simulink model "power_system"  (R2026b)
settings: Solver=VariableStepAuto  StopTime=param.sim.simlength
model workspace (MAT data in the model file):
  phi = 0.785398163397
values from neighbouring files (symbols this model uses):
  param = struct()    [init_model.m]
undefined symbols (not defined in the file or in its folder): dmavg_flt, simple_moving_average_filter
libraries: fl_lib x37, nesl_utility x22, single_phase_transformer_lib x3, saturable_single_phase_transformer x3, power_meter_iec x2, three_phase_transformer_lib x2, eeGeneralControl x2, moving_average_filter x1, moving_average_filter_cc x1, simulink x1, three_phase_voltage_with_frt_emulator x1, three_phase_rl_load x1
(part 2 of 2)

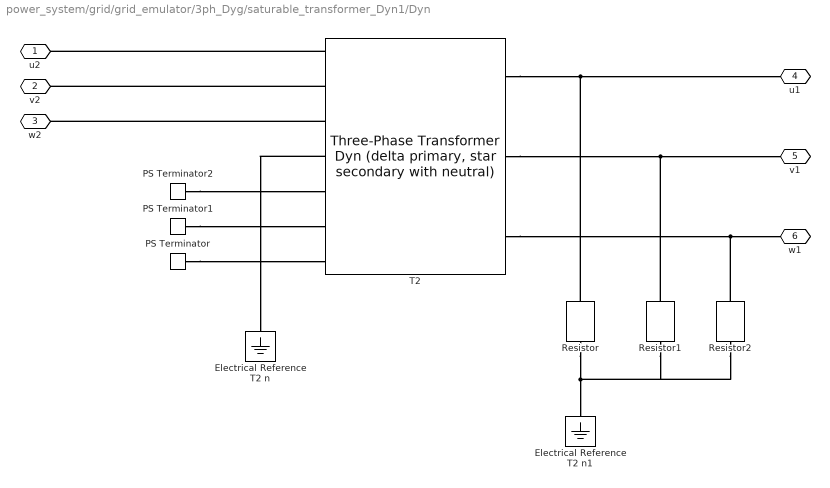
== system power_system/grid/grid_emulator/3ph_Dyg/saturable_transformer_Dyn1/Dyn ==
  Electrical Reference T2 n : fl_lib/Electrical/Electrical Elements/Electrical Reference
  Electrical Reference T2 n1 : fl_lib/Electrical/Electrical Elements/Electrical Reference
  PS Terminator : fl_lib/Physical Signals/Sinks/PS Terminator
  PS Terminator1 : fl_lib/Physical Signals/Sinks/PS Terminator
  PS Terminator2 : fl_lib/Physical Signals/Sinks/PS Terminator
  Resistor : fl_lib/Electrical/Electrical Elements/Resistor  R=1e4 Ohm  i_specify=off  i_priority=None  i=0 A  i_nominal_specify=off  i_nominal_value=1  i_nominal_unit=A  v_specify=off  v_priority=None  v=0 V  v_nominal_specify=off  v_nominal_value=1  v_nominal_unit=V
  Resistor1 : fl_lib/Electrical/Electrical Elements/Resistor  R=1e4 Ohm  i_specify=off  i_priority=None  i=0 A  i_nominal_specify=off  i_nominal_value=1  i_nominal_unit=A  v_specify=off  v_priority=None  v=0 V  v_nominal_specify=off  v_nominal_value=1  v_nominal_unit=V
  Resistor2 : fl_lib/Electrical/Electrical Elements/Resistor  R=1e4 Ohm  i_specify=off  i_priority=None  i=0 A  i_nominal_specify=off  i_nominal_value=1  i_nominal_unit=A  v_specify=off  v_priority=None  v=0 V  v_nominal_specify=off  v_nominal_value=1  v_nominal_unit=V
  T2 : three_phase_transformer_lib/Three-Phase Transformer Dyn (delta primary, star secondary with neutral)  Sr=param.load.trafo.pu.Sr A*V  V1=param.load.trafo.pu.V1 V  V2=param.load.trafo.pu.V2 V  fr=param.load.trafo.pu.fr Hz  clock_number=param.load.trafo.pu.clock  r1=param.load.trafo.pu.r1  l1=param.load.trafo.pu.l1  r2=param.load.trafo.pu.r2  l2=param.load.trafo.pu.l2  lm=param.load.trafo.pu.lm  lm0=param.load.trafo.pu.lm0  rfe=param.load.trafo.pu.rfe  iAB_specify=off  iAB_priority=None  iAB=0 A  iAB_nominal_specify=off  iAB_nominal_value=1  iAB_nominal_unit=A  iBC_specify=off  iBC_priority=None  iBC=0 A  iBC_nominal_specify=off  iBC_nominal_value=1  iBC_nominal_unit=A  iCA_specify=off  iCA_priority=None  iCA=0 A  iCA_nominal_specify=off  iCA_nominal_value=1  iCA_nominal_unit=A  i2a_specify=off  i2a_priority=None  i2a=0 A  i2a_nominal_specify=off  i2a_nominal_value=1  i2a_nominal_unit=A  i2b_specify=off  i2b_priority=None  i2b=0 A  i2b_nominal_specify=off  i2b_nominal_value=1  i2b_nominal_unit=A  i2c_specify=off  i2c_priority=None  i2c=0 A  i2c_nominal_specify=off  i2c_nominal_value=1  i2c_nominal_unit=A
  u2 : PMIOPort  Side=Left
  v2 : PMIOPort  Port=2  Side=Left
  w2 : PMIOPort  Port=3  Side=Left
  u1 : PMIOPort  Port=4  Side=Right
  v1 : PMIOPort  Port=5  Side=Right
  w1 : PMIOPort  Port=6  Side=Right
  connections:
  PS Terminator2/LConn1 -- T2/RConn5
  T2/RConn3 -- w2/RConn1
  T2/RConn4 -- Electrical Reference T2 n/LConn1
  PS Terminator1/LConn1 -- T2/RConn6
  T2/LConn1 -- Resistor/LConn1 -- u1/RConn1
  T2/LConn2 -- Resistor1/LConn1 -- v1/RConn1
  T2/LConn3 -- Resistor2/LConn1 -- w1/RConn1
  T2/RConn1 -- u2/RConn1
  PS Terminator/LConn1 -- T2/RConn7
  T2/RConn2 -- v2/RConn1
  Resistor/RConn1 -- Resistor2/RConn1 -- Resistor1/RConn1 -- Electrical Reference T2 n1/LConn1

== matlab function power_system/analysis/moving average filters1/dyn_mavg1/dyn_mavg ==
  data: input input; period input; ts input; y output
function y = mavgflt_process(input, period, ts)
%#codegen
% MAVGFLT_PROCESS  Moving Average Filter con periodo variabile e frazionario
%
%   y = mavgflt_process(input, period, ts)
%
%   Filtro a media mobile con:
%   - Buffer circolare
%   - Periodo variabile e frazionario
%   - Aggiornamento incrementale (alta efficienza)
%
%   Compatibile con Simulink (persistent variables)
%   ts (s) : sampling time
%   period (s) : periodo su cui si vuole fare la media
%   input : segnale da mediare.

    % Parametri fissi
    MAVGFLT_SIZE_MAX = 1750; % MAVGFLT_SIZE_MAX > di 200ms/125us

    % Variabili persistenti (mantengono lo stato tra chiamate)
    persistent buffer cb_index sample_count sum_short sum_long prev_input

    % Inizializzazione al primo passo
    if isempty(buffer)
        buffer       = zeros(1, MAVGFLT_SIZE_MAX); %vettore del buffer circolare (1×MAVGFLT_SIZE_MAX)
        cb_index     = 1;   % current buffer index: indice di scrittura corrente
        sample_count = 1;   % sample count : numero di campioni attivi nella finestra, questo
                            % (e il suo sample_count-1) è il numero di
                            % campioni con cui farò la media.
                            % sample_count parte da zero e man mano cresce
                            % e viene aumentato e contratto a seconda del
                            % valore di n_samples.
        sum_short    = 0;   % somma corta
        sum_long     = 0;   % somma lunga
        prev_input   = 0;   % ultimo valore di ingresso 
    end

    % Gestione caso periodo nullo o negativo
    if period <= 0
        y = 0;
        return;
    end

    % Numero desiderato di campioni: è un nemero reale
    desired_samples = period / ts;

    % Limite massimo
    if desired_samples > (MAVGFLT_SIZE_MAX - 1)
        desired_samples = MAVGFLT_SIZE_MAX - 1;
    end

    % Parte intera e frazionaria
    % es: 
    % desired_samples = 20.8
    % n_samples = 21
    % frac = 0.8
    % desired_samples = 20.2
    % n_samples = 21
    % frac = 0.2
    n_samples = floor(desired_samples + 1); % numero di campioni che coprono interamente il periodo
    frac = desired_samples + 1 - n_samples; % parte prazionaria 

    % Evita finestre vuote
    if n_samples < 1
        n_samples = 1;
    end

    % --- Aggiornamento somme ---
    if n_samples > sample_count
        % Finestra aumenta → aggiungi nuovi campioni
        sum_short = sum_short + prev_input;
        sum_long  = sum_long  + input;
        sample_count = sample_count + 1;

    elseif n_samples < sample_count
        % Finestra ridotta → rimuovi i campioni più vecchi
        oldest1 = buffer_index(cb_index, sample_count, MAVGFLT_SIZE_MAX);
        oldest2 = buffer_index(cb_index, sample_count - 1, MAVGFLT_SIZE_MAX);

        oldest_sum = buffer(oldest1) + buffer(oldest2);

        sum_short = sum_short + prev_input - oldest_sum;
        sum_long  = sum_long  + input - oldest_sum;

        sample_count = sample_count - 1;

    else
        % Finestra costante
        oldest = buffer_value(buffer, cb_index, sample_count, MAVGFLT_SIZE_MAX);
        sum_short = sum_short + prev_input - oldest;
        sum_long  = sum_long  + input - oldest;
    end

    % --- Aggiornamento buffer circolare ---
    buffer(cb_index) = input;
    cb_index = mod(cb_index, MAVGFLT_SIZE_MAX) + 1;
    prev_input = input;

    % --- Calcolo output ---
    if sample_count > 1
        avg_short = sum_short / (sample_count - 1);
    else
        avg_short = 0;
    end
    avg_long = sum_long / sample_count;

    % Interpolazione lineare tra finestre
    y = avg_short * (1 - frac) + avg_long * frac;
end


% =====================================================================
function idx = buffer_index(cb_index, offset, max_size)
% Calcola indice 1-based di un campione "offset" passi indietro nel buffer
% circolare
    idx = mod(cb_index - 1 - offset, max_size) + 1;
end

function val = buffer_value(buffer, cb_index, offset, max_size)
% Restituisce il valore del buffer "offset" passi indietro
    idx = mod(cb_index - 1 - offset, max_size) + 1;
    val = buffer(idx);
end
